simulink model "Read_OpticalFlow_Record"  (R2021b)
settings: Solver=ode2  StartTime=0.0  StopTime=inf  FixedStep=0.001  RelTol=1e-3  EnableMultiTasking=on
model workspace (MAT data in the model file):
  target_system = 1
undefined symbols (not defined in the file): gcbh, JPEG, qc_get_step_size, Video3D, video_display_show
libraries: quarc_library x29
settings Model: SimulationMode=external  ExtModeTrigDuration=10000  Creator=dmadill  LastModifiedBy=user
settings SolverCC: AlgebraicLoopSolver=TrustRegion  PositivePriorityOrder=on
settings DataIOCC: LimitDataPoints=on  SaveFormat=Array  ReturnWorkspaceOutputs=off
settings DebuggingCC: SolverPrmCheckMsg=warning  SFUnexpectedBacktrackingDiag=warning  SFNoUnconditionalDefaultTransitionDiag=warning  SFExecutionAtInitializationDiag=none  SFMachineParentedDataDiag=warning  ArithmeticOperatorsInVariantConditions=warning
settings HardwareCC: ProdBitPerLong=64  ProdHWDeviceType=Intel->x86-64 (Linux 64)
settings ModelReferenceCC: PropagateSignalLabelsOutOfModel=off
settings SFSimCC: SimUseLocalCustomCode=off  CustomCodeUndefinedFunction=UseInterfaceOnly
settings RTWCC: Description=QUARC Linux x64 Target (QDrone) Using Toolchain  SystemTargetFile=quarc_linux_x64.tlc  TemplateMakefile=quarc_default_tmf  RTWUseLocalCustomCode=off  Toolchain=QUARC linux_x64 | gmake (64-bit Windows)  BuildConfiguration=Faster Runs
settings CodeAppCC: StateflowObjectComments=on
settings STFCustomTargetCC: ConcurrentExecutionCompliant=on  UseToolchainInfoCompliant=on  SystemTargetFile=quarc_linux_x64.tlc
settings GRTTargetCC: TargetLangStandard=C89/C90 (ANSI)  ParMdlRefBuildCompliant=off  CompOptLevelCompliant=off  CombineOutputUpdateFcns=off  MatFileLogging=off  CPPClassGenCompliant=off  GRTInterface=on  ExtMode=on  ExtModeMexFile=quarc_comm  ExtModeMexArgs='-w -d /tmp -uri %u', 'tcpip://192.168.2.15:17002?retries=10'
settings ConfigComp: CovMetricSettings=dw  CovSaveCumulativeToWorkspaceVar=on  CovSaveSingleToWorkspaceVar=on  CovExternalEMLEnable=off  CovSFcnEnable=off

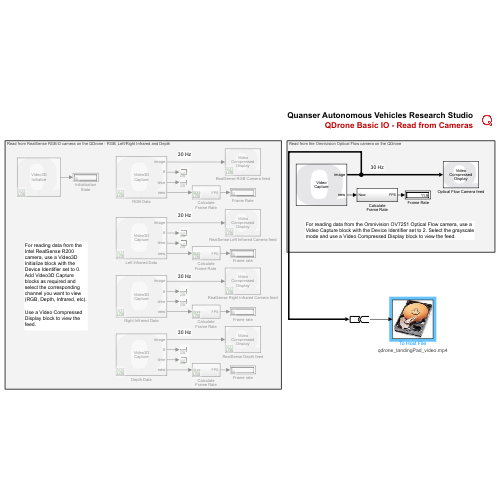
[thumbnail: Simulink's stored preview of the top-level diagram]
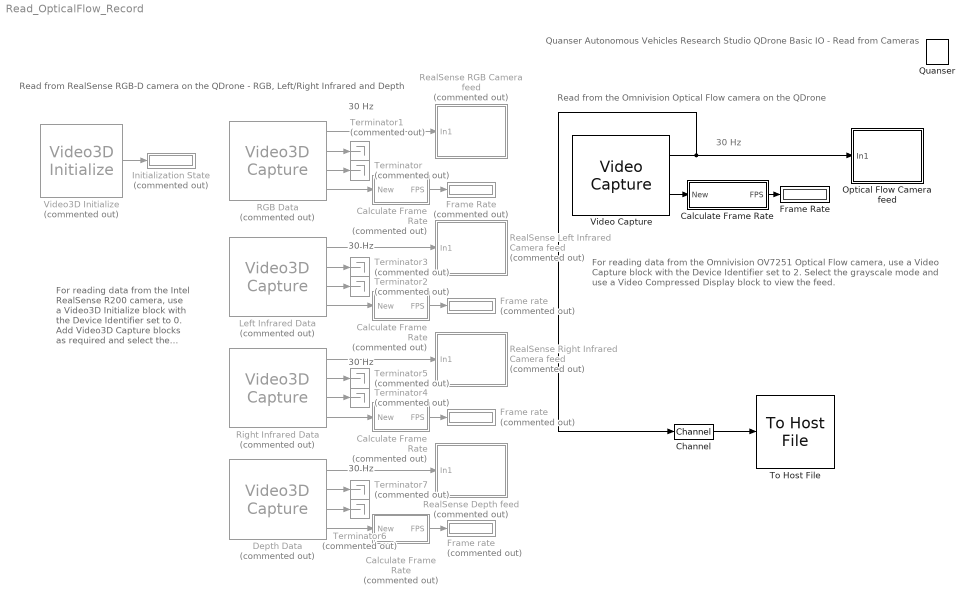
== system Read_OpticalFlow_Record ==
  note: 30 Hz
  note: For reading data from the Omnivision OV7251 Optical Flow camera, use a
      | Video Capture block with the Device Identifier set to 2. Select the grayscale
      | mode and use a Video Compressed Display block to view the feed.
  note: For reading data from the Intel RealSense R200 camera, use a Video3D Initialize block with the Device Identifier set to 0. Add Video3D Capture blocks as required and select the corresponding channel you want to view (RGB, Depth, Infrared, etc).
      |
      | Use a Video Compressed Display block to view the feed.
  note: Read from the Omnivision Optical Flow camera on the QDrone
  note: Read from RealSense RGB-D camera on the QDrone - RGB, Left/Right Infrared and Depth
  note: Quanser Autonomous Vehicles Research Studio
      | QDrone Basic IO - Read from Cameras
  note: 30 Hz
  note: 30 Hz
  note: 30 Hz
  note: 30 Hz
  "   Frame rate   " : Display  Commented=on
  "  Frame Rate " : Display
  "  Frame rate  " : Display  Commented=on
  " Calculate Frame Rate" : Subsystem
  " Frame rate " : Display  Commented=on
  "Calculate Frame Rate  " : Subsystem  Commented=on
  "Calculate Frame Rate " : Subsystem  Commented=on
  Calculate Frame Rate : Subsystem  Commented=on
  "Calculate Frame Rate " : Subsystem  Commented=on
  Channel : quarc_library/Signal Routing/Channel  channel=0  buffer_size=1
  Depth Data : quarc_library/Multimedia/Video3D Capture  Commented=on  object_name=unassigned  stream_type=Depth  stream_index=0  resolution=640 x 480  width=640  height=480  output_format=MATLAB greyscale (HxW)  data_type=uint16  sample_time=qc_get_step_size * ceil(0.033 / qc_get_step_size)  camera_intrinsics=off  depth_scale=off  brightness_override=off  brightness=50.0  contrast_override=off  contrast=50.0  hue_override=off  hue=50.0  saturation_override=off  saturation=50.0  sharpness_override=off  sharpness=50.0  gamma_override=off  gamma=50.0  gain_override=off  gain=50.0  backlightcompensation_override=off  backlightcompensation=50.0  whitebalance_override=Automatic white balance  whitebalance=50.0  exposure_override=Automatic exposure  exposure=30.0  emitter=Enable laser emitter  preset=Do not set camera presets
  Frame Rate : Display  Commented=on
  Initialization State : Display  Commented=on
  Left Infrared Data : quarc_library/Multimedia/Video3D Capture  Commented=on  object_name=unassigned  stream_type=Infrared  stream_index=0  resolution=640 x 480  width=640  height=480  output_format=MATLAB greyscale (HxW)  data_type=uint8  sample_time=qc_get_step_size * ceil(0.033 / qc_get_step_size)  camera_intrinsics=off  depth_scale=off  brightness_override=off  brightness=50.0  contrast_override=off  contrast=50.0  hue_override=off  hue=50.0  saturation_override=off  saturation=50.0  sharpness_override=off  sharpness=50.0  gamma_override=off  gamma=50.0  gain_override=off  gain=50.0  backlightcompensation_override=off  backlightcompensation=50.0  whitebalance_override=Automatic white balance  whitebalance=50.0  exposure_override=Automatic exposure  exposure=30.0  emitter=Enable laser emitter  preset=Do not set camera presets
  Optical Flow Camera feed : Subsystem  LoadFcn=set_param(gcbh, 'UserData', gcb);  StartFcn=video_display_show([gcb, '/Video Display'], 'add', gcb);  mask(Video Compressed Display){algorithm=JPEG, quality=50, sample_time=-1, use_hardware=on}
      mask prompts: algorithm "Compression algorithm:"; quality "Compression quality (0-100):"; sample_time "Sample time (seconds):"; use_hardware "Use hardware acceleration for video display"
      mask help: Displays a video stream on the host, using compression to minimize bandwidth.
      mask init:
      | qc_set_display('Video\nCompressed\nDisplay');
      settings: UndoDeleteFcn=set_param(gcbh, 'UserData', gcb);  OpenFcn=video_display_show([gcb, '/Video Display'], 'show', gcb);  PreDeleteFcn=video_display_show([gcb, '/Video Display'], 'delete');
      settings: CopyFcn=|
      | set_param(gcbh, 'UserData', gcb);
      | set_param(gcbh, 'LinkStatus', 'none');
      settings: NameChangeFcn=|
      | video_display_show([get_param(gcbh, 'UserData'), '/Video Display'], 'rename', [gcb, '/Video Display']);
      | video_display_show([gcb, '/Video Display'], 'add', gcb);
      | set_param(gcbh, 'UserData', gcb);
      mask Help: web(qc_get_block_help_path(gcb));
      mask TypeOptions algorithm: Image Compress/algorithm
      mask TypeOptions quality: Image Compress/quality
      mask TypeOptions sample_time: Video Display/sample_time
      mask TypeOptions use_hardware: Video Display/use_hardware
      mask Display:
      | patch([0.98591 0.98591 0.62618 0.59072 0.56147   0.536   0.536  0.5441 0.56912 0.59207 0.60881 0.62276 0.63527 0.64364  0.6485  0.6485 0.64706 0.64499 0.63662 0.62411 0.61232 0.59837 0.58307 0.56147   0.536   0.536  0.5441  0.5747 0.60953 0.63662 0.67001  0.7034 0.72851 0.75425 0.77927 0.80294 0.82454 0.84119 0.85865 0.87395 0.88574 0.89339  0.8969 0.89969 0.89969 0.89267  0.8816 0.87044 0.85649  0.8384 0.81824 0.80294 0.78764 0.77513 0.76676 0.75776 0.76397 0.77513 0.79178 0.80987 0.82796 0.84326 0.86207 0.98528],[0.18689 0.05522 0.05522 0.05171 0.05171    0.05 0.18338 0.18338 0.19148 0.20435 0.22298 0.24863 0.28589 0.33125 0.38138 0.55139 0.59801 0.63761 0.68189 0.72149 0.74939 0.76694 0.77855 0.79367 0.79952 0.92768 0.92768 0.92768 0.92417 0.92066 0.91364  0.9032 0.89384 0.88106 0.86594 0.85073 0.82634 0.80537 0.77855 0.74363 0.70403 0.65858 0.61079 0.59099 0.41513 0.37202 0.31847 0.29048 0.25556 0.23342  0.2102 0.19382 0.18221 0.17285 0.16943 0.16124  0.1589 0.16241 0.16709 0.17168  0.1787 0.18221 0.18689 0.18689],[0.9,0.90,0.91])
      | patch([0.536 0.52601 0.46823 0.44528 0.41603 0.39101 0.35555 0.33116 0.31451 0.29291  0.2804 0.26717 0.25322 0.23999 0.22406 0.20732 0.19337 0.17528 0.15935 0.14396 0.13217 0.11759 0.10922 0.10085 0.09671 0.09392 0.09041 0.08906 0.08906 0.09464  0.0995 0.10778 0.11894 0.13145 0.14675 0.16349 0.17672 0.19409 0.20732 0.22406 0.23999 0.26159 0.27833 0.29849 0.31793 0.33602 0.35411 0.37085 0.39245 0.41603   0.536   0.536 0.53159 0.46409   0.446 0.42026 0.39587 0.37571 0.36113 0.34925 0.34088 0.33809 0.33809 0.34088 0.34583 0.35627 0.36392 0.38129 0.39587 0.41117 0.42719 0.44672  0.4676 0.48353 0.48353 0.52394   0.536],[0.05 0.04829 0.04712 0.04712 0.04829 0.05063 0.05405 0.05873 0.06107 0.06692 0.07043 0.07619 0.08087 0.08672 0.09482 0.10652 0.11696 0.13325  0.1508 0.17168 0.19499 0.22415 0.25439 0.28472 0.31379 0.35456 0.38489 0.41513 0.58055 0.63878 0.68774 0.72149 0.75641 0.78089 0.80537 0.82859 0.84029 0.85658 0.86594 0.87404  0.8834 0.89267 0.90086 0.90788 0.91247 0.91832 0.92066   0.923 0.92651 0.92768 0.92768 0.79952 0.79952 0.79952 0.79718 0.78899 0.77153 0.75056 0.72149 0.68072 0.62249  0.5549 0.41396 0.37085 0.33242 0.28121 0.25205 0.22181 0.20552 0.19499 0.18572 0.18221 0.17753 0.17636 0.17753  0.1787  0.1787],[0.9,0.90,0.91])
      | disp('Video\nCompressed\nDisplay');
  Quanser : quarc_library/Logos/Quanser
  RGB Data : quarc_library/Multimedia/Video3D Capture  Commented=on  object_name=unassigned  stream_type=RGB  stream_index=0  resolution=640 x 480  width=640  height=480  output_format=MATLAB RGB (HxWx3)  data_type=uint8  sample_time=qc_get_step_size * ceil(0.033 / qc_get_step_size)  camera_intrinsics=off  depth_scale=off  brightness_override=off  brightness=50.0  contrast_override=off  contrast=50.0  hue_override=off  hue=50.0  saturation_override=off  saturation=50.0  sharpness_override=off  sharpness=50.0  gamma_override=off  gamma=50.0  gain_override=off  gain=50.0  backlightcompensation_override=off  backlightcompensation=50.0  whitebalance_override=Automatic white balance  whitebalance=50.0  exposure_override=Automatic exposure  exposure=30.0  emitter=Enable laser emitter  preset=Do not set camera presets
  RealSense Depth feed : Subsystem  Commented=on  LoadFcn=set_param(gcbh, 'UserData', gcb);  StartFcn=video_display_show([gcb, '/Video Display'], 'add', gcb);  mask(Video Compressed Display){algorithm=JPEG, quality=50, sample_time=-1, use_hardware=on}
      mask prompts: algorithm "Compression algorithm:"; quality "Compression quality (0-100):"; sample_time "Sample time (seconds):"; use_hardware "Use hardware acceleration for video display"
      mask help: Displays a video stream on the host, using compression to minimize bandwidth.
      mask init:
      | qc_set_display('Video\nCompressed\nDisplay');
      settings: UndoDeleteFcn=set_param(gcbh, 'UserData', gcb);  OpenFcn=video_display_show([gcb, '/Video Display'], 'show', gcb);  PreDeleteFcn=video_display_show([gcb, '/Video Display'], 'delete');
      settings: CopyFcn=|
      | set_param(gcbh, 'UserData', gcb);
      | set_param(gcbh, 'LinkStatus', 'none');
      settings: NameChangeFcn=|
      | video_display_show([get_param(gcbh, 'UserData'), '/Video Display'], 'rename', [gcb, '/Video Display']);
      | video_display_show([gcb, '/Video Display'], 'add', gcb);
      | set_param(gcbh, 'UserData', gcb);
      mask Help: web(qc_get_block_help_path(gcb));
      mask TypeOptions algorithm: Image Compress/algorithm
      mask TypeOptions quality: Image Compress/quality
      mask TypeOptions sample_time: Video Display/sample_time
      mask TypeOptions use_hardware: Video Display/use_hardware
      mask Display:
      | patch([0.98591 0.98591 0.62618 0.59072 0.56147   0.536   0.536  0.5441 0.56912 0.59207 0.60881 0.62276 0.63527 0.64364  0.6485  0.6485 0.64706 0.64499 0.63662 0.62411 0.61232 0.59837 0.58307 0.56147   0.536   0.536  0.5441  0.5747 0.60953 0.63662 0.67001  0.7034 0.72851 0.75425 0.77927 0.80294 0.82454 0.84119 0.85865 0.87395 0.88574 0.89339  0.8969 0.89969 0.89969 0.89267  0.8816 0.87044 0.85649  0.8384 0.81824 0.80294 0.78764 0.77513 0.76676 0.75776 0.76397 0.77513 0.79178 0.80987 0.82796 0.84326 0.86207 0.98528],[0.18689 0.05522 0.05522 0.05171 0.05171    0.05 0.18338 0.18338 0.19148 0.20435 0.22298 0.24863 0.28589 0.33125 0.38138 0.55139 0.59801 0.63761 0.68189 0.72149 0.74939 0.76694 0.77855 0.79367 0.79952 0.92768 0.92768 0.92768 0.92417 0.92066 0.91364  0.9032 0.89384 0.88106 0.86594 0.85073 0.82634 0.80537 0.77855 0.74363 0.70403 0.65858 0.61079 0.59099 0.41513 0.37202 0.31847 0.29048 0.25556 0.23342  0.2102 0.19382 0.18221 0.17285 0.16943 0.16124  0.1589 0.16241 0.16709 0.17168  0.1787 0.18221 0.18689 0.18689],[0.9,0.90,0.91])
      | patch([0.536 0.52601 0.46823 0.44528 0.41603 0.39101 0.35555 0.33116 0.31451 0.29291  0.2804 0.26717 0.25322 0.23999 0.22406 0.20732 0.19337 0.17528 0.15935 0.14396 0.13217 0.11759 0.10922 0.10085 0.09671 0.09392 0.09041 0.08906 0.08906 0.09464  0.0995 0.10778 0.11894 0.13145 0.14675 0.16349 0.17672 0.19409 0.20732 0.22406 0.23999 0.26159 0.27833 0.29849 0.31793 0.33602 0.35411 0.37085 0.39245 0.41603   0.536   0.536 0.53159 0.46409   0.446 0.42026 0.39587 0.37571 0.36113 0.34925 0.34088 0.33809 0.33809 0.34088 0.34583 0.35627 0.36392 0.38129 0.39587 0.41117 0.42719 0.44672  0.4676 0.48353 0.48353 0.52394   0.536],[0.05 0.04829 0.04712 0.04712 0.04829 0.05063 0.05405 0.05873 0.06107 0.06692 0.07043 0.07619 0.08087 0.08672 0.09482 0.10652 0.11696 0.13325  0.1508 0.17168 0.19499 0.22415 0.25439 0.28472 0.31379 0.35456 0.38489 0.41513 0.58055 0.63878 0.68774 0.72149 0.75641 0.78089 0.80537 0.82859 0.84029 0.85658 0.86594 0.87404  0.8834 0.89267 0.90086 0.90788 0.91247 0.91832 0.92066   0.923 0.92651 0.92768 0.92768 0.79952 0.79952 0.79952 0.79718 0.78899 0.77153 0.75056 0.72149 0.68072 0.62249  0.5549 0.41396 0.37085 0.33242 0.28121 0.25205 0.22181 0.20552 0.19499 0.18572 0.18221 0.17753 0.17636 0.17753  0.1787  0.1787],[0.9,0.90,0.91])
      | disp('Video\nCompressed\nDisplay');
  RealSense Left Infrared Camera feed : Subsystem  Commented=on  LoadFcn=set_param(gcbh, 'UserData', gcb);  StartFcn=video_display_show([gcb, '/Video Display'], 'add', gcb);  mask(Video Compressed Display){algorithm=JPEG, quality=50, sample_time=-1, use_hardware=on}
      mask prompts: algorithm "Compression algorithm:"; quality "Compression quality (0-100):"; sample_time "Sample time (seconds):"; use_hardware "Use hardware acceleration for video display"
      mask help: Displays a video stream on the host, using compression to minimize bandwidth.
      mask init:
      | qc_set_display('Video\nCompressed\nDisplay');
      settings: UndoDeleteFcn=set_param(gcbh, 'UserData', gcb);  OpenFcn=video_display_show([gcb, '/Video Display'], 'show', gcb);  PreDeleteFcn=video_display_show([gcb, '/Video Display'], 'delete');
      settings: CopyFcn=|
      | set_param(gcbh, 'UserData', gcb);
      | set_param(gcbh, 'LinkStatus', 'none');
      settings: NameChangeFcn=|
      | video_display_show([get_param(gcbh, 'UserData'), '/Video Display'], 'rename', [gcb, '/Video Display']);
      | video_display_show([gcb, '/Video Display'], 'add', gcb);
      | set_param(gcbh, 'UserData', gcb);
      mask Help: web(qc_get_block_help_path(gcb));
      mask TypeOptions algorithm: Image Compress/algorithm
      mask TypeOptions quality: Image Compress/quality
      mask TypeOptions sample_time: Video Display/sample_time
      mask TypeOptions use_hardware: Video Display/use_hardware
      mask Display:
      | patch([0.98591 0.98591 0.62618 0.59072 0.56147   0.536   0.536  0.5441 0.56912 0.59207 0.60881 0.62276 0.63527 0.64364  0.6485  0.6485 0.64706 0.64499 0.63662 0.62411 0.61232 0.59837 0.58307 0.56147   0.536   0.536  0.5441  0.5747 0.60953 0.63662 0.67001  0.7034 0.72851 0.75425 0.77927 0.80294 0.82454 0.84119 0.85865 0.87395 0.88574 0.89339  0.8969 0.89969 0.89969 0.89267  0.8816 0.87044 0.85649  0.8384 0.81824 0.80294 0.78764 0.77513 0.76676 0.75776 0.76397 0.77513 0.79178 0.80987 0.82796 0.84326 0.86207 0.98528],[0.18689 0.05522 0.05522 0.05171 0.05171    0.05 0.18338 0.18338 0.19148 0.20435 0.22298 0.24863 0.28589 0.33125 0.38138 0.55139 0.59801 0.63761 0.68189 0.72149 0.74939 0.76694 0.77855 0.79367 0.79952 0.92768 0.92768 0.92768 0.92417 0.92066 0.91364  0.9032 0.89384 0.88106 0.86594 0.85073 0.82634 0.80537 0.77855 0.74363 0.70403 0.65858 0.61079 0.59099 0.41513 0.37202 0.31847 0.29048 0.25556 0.23342  0.2102 0.19382 0.18221 0.17285 0.16943 0.16124  0.1589 0.16241 0.16709 0.17168  0.1787 0.18221 0.18689 0.18689],[0.9,0.90,0.91])
      | patch([0.536 0.52601 0.46823 0.44528 0.41603 0.39101 0.35555 0.33116 0.31451 0.29291  0.2804 0.26717 0.25322 0.23999 0.22406 0.20732 0.19337 0.17528 0.15935 0.14396 0.13217 0.11759 0.10922 0.10085 0.09671 0.09392 0.09041 0.08906 0.08906 0.09464  0.0995 0.10778 0.11894 0.13145 0.14675 0.16349 0.17672 0.19409 0.20732 0.22406 0.23999 0.26159 0.27833 0.29849 0.31793 0.33602 0.35411 0.37085 0.39245 0.41603   0.536   0.536 0.53159 0.46409   0.446 0.42026 0.39587 0.37571 0.36113 0.34925 0.34088 0.33809 0.33809 0.34088 0.34583 0.35627 0.36392 0.38129 0.39587 0.41117 0.42719 0.44672  0.4676 0.48353 0.48353 0.52394   0.536],[0.05 0.04829 0.04712 0.04712 0.04829 0.05063 0.05405 0.05873 0.06107 0.06692 0.07043 0.07619 0.08087 0.08672 0.09482 0.10652 0.11696 0.13325  0.1508 0.17168 0.19499 0.22415 0.25439 0.28472 0.31379 0.35456 0.38489 0.41513 0.58055 0.63878 0.68774 0.72149 0.75641 0.78089 0.80537 0.82859 0.84029 0.85658 0.86594 0.87404  0.8834 0.89267 0.90086 0.90788 0.91247 0.91832 0.92066   0.923 0.92651 0.92768 0.92768 0.79952 0.79952 0.79952 0.79718 0.78899 0.77153 0.75056 0.72149 0.68072 0.62249  0.5549 0.41396 0.37085 0.33242 0.28121 0.25205 0.22181 0.20552 0.19499 0.18572 0.18221 0.17753 0.17636 0.17753  0.1787  0.1787],[0.9,0.90,0.91])
      | disp('Video\nCompressed\nDisplay');
  RealSense RGB Camera feed : Subsystem  Commented=on  LoadFcn=set_param(gcbh, 'UserData', gcb);  StartFcn=video_display_show([gcb, '/Video Display'], 'add', gcb);  mask(Video Compressed Display){algorithm=JPEG, quality=50, sample_time=-1, use_hardware=on}
      mask prompts: algorithm "Compression algorithm:"; quality "Compression quality (0-100):"; sample_time "Sample time (seconds):"; use_hardware "Use hardware acceleration for video display"
      mask help: Displays a video stream on the host, using compression to minimize bandwidth.
      mask init:
      | qc_set_display('Video\nCompressed\nDisplay');
      settings: UndoDeleteFcn=set_param(gcbh, 'UserData', gcb);  OpenFcn=video_display_show([gcb, '/Video Display'], 'show', gcb);  PreDeleteFcn=video_display_show([gcb, '/Video Display'], 'delete');
      settings: CopyFcn=|
      | set_param(gcbh, 'UserData', gcb);
      | set_param(gcbh, 'LinkStatus', 'none');
      settings: NameChangeFcn=|
      | video_display_show([get_param(gcbh, 'UserData'), '/Video Display'], 'rename', [gcb, '/Video Display']);
      | video_display_show([gcb, '/Video Display'], 'add', gcb);
      | set_param(gcbh, 'UserData', gcb);
      mask Help: web(qc_get_block_help_path(gcb));
      mask TypeOptions algorithm: Image Compress/algorithm
      mask TypeOptions quality: Image Compress/quality
      mask TypeOptions sample_time: Video Display/sample_time
      mask TypeOptions use_hardware: Video Display/use_hardware
      mask Display:
      | patch([0.98591 0.98591 0.62618 0.59072 0.56147   0.536   0.536  0.5441 0.56912 0.59207 0.60881 0.62276 0.63527 0.64364  0.6485  0.6485 0.64706 0.64499 0.63662 0.62411 0.61232 0.59837 0.58307 0.56147   0.536   0.536  0.5441  0.5747 0.60953 0.63662 0.67001  0.7034 0.72851 0.75425 0.77927 0.80294 0.82454 0.84119 0.85865 0.87395 0.88574 0.89339  0.8969 0.89969 0.89969 0.89267  0.8816 0.87044 0.85649  0.8384 0.81824 0.80294 0.78764 0.77513 0.76676 0.75776 0.76397 0.77513 0.79178 0.80987 0.82796 0.84326 0.86207 0.98528],[0.18689 0.05522 0.05522 0.05171 0.05171    0.05 0.18338 0.18338 0.19148 0.20435 0.22298 0.24863 0.28589 0.33125 0.38138 0.55139 0.59801 0.63761 0.68189 0.72149 0.74939 0.76694 0.77855 0.79367 0.79952 0.92768 0.92768 0.92768 0.92417 0.92066 0.91364  0.9032 0.89384 0.88106 0.86594 0.85073 0.82634 0.80537 0.77855 0.74363 0.70403 0.65858 0.61079 0.59099 0.41513 0.37202 0.31847 0.29048 0.25556 0.23342  0.2102 0.19382 0.18221 0.17285 0.16943 0.16124  0.1589 0.16241 0.16709 0.17168  0.1787 0.18221 0.18689 0.18689],[0.9,0.90,0.91])
      | patch([0.536 0.52601 0.46823 0.44528 0.41603 0.39101 0.35555 0.33116 0.31451 0.29291  0.2804 0.26717 0.25322 0.23999 0.22406 0.20732 0.19337 0.17528 0.15935 0.14396 0.13217 0.11759 0.10922 0.10085 0.09671 0.09392 0.09041 0.08906 0.08906 0.09464  0.0995 0.10778 0.11894 0.13145 0.14675 0.16349 0.17672 0.19409 0.20732 0.22406 0.23999 0.26159 0.27833 0.29849 0.31793 0.33602 0.35411 0.37085 0.39245 0.41603   0.536   0.536 0.53159 0.46409   0.446 0.42026 0.39587 0.37571 0.36113 0.34925 0.34088 0.33809 0.33809 0.34088 0.34583 0.35627 0.36392 0.38129 0.39587 0.41117 0.42719 0.44672  0.4676 0.48353 0.48353 0.52394   0.536],[0.05 0.04829 0.04712 0.04712 0.04829 0.05063 0.05405 0.05873 0.06107 0.06692 0.07043 0.07619 0.08087 0.08672 0.09482 0.10652 0.11696 0.13325  0.1508 0.17168 0.19499 0.22415 0.25439 0.28472 0.31379 0.35456 0.38489 0.41513 0.58055 0.63878 0.68774 0.72149 0.75641 0.78089 0.80537 0.82859 0.84029 0.85658 0.86594 0.87404  0.8834 0.89267 0.90086 0.90788 0.91247 0.91832 0.92066   0.923 0.92651 0.92768 0.92768 0.79952 0.79952 0.79952 0.79718 0.78899 0.77153 0.75056 0.72149 0.68072 0.62249  0.5549 0.41396 0.37085 0.33242 0.28121 0.25205 0.22181 0.20552 0.19499 0.18572 0.18221 0.17753 0.17636 0.17753  0.1787  0.1787],[0.9,0.90,0.91])
      | disp('Video\nCompressed\nDisplay');
  RealSense Right Infrared Camera feed : Subsystem  Commented=on  LoadFcn=set_param(gcbh, 'UserData', gcb);  StartFcn=video_display_show([gcb, '/Video Display'], 'add', gcb);  mask(Video Compressed Display){algorithm=JPEG, quality=50, sample_time=-1, use_hardware=on}
      mask prompts: algorithm "Compression algorithm:"; quality "Compression quality (0-100):"; sample_time "Sample time (seconds):"; use_hardware "Use hardware acceleration for video display"
      mask help: Displays a video stream on the host, using compression to minimize bandwidth.
      mask init:
      | qc_set_display('Video\nCompressed\nDisplay');
      settings: UndoDeleteFcn=set_param(gcbh, 'UserData', gcb);  OpenFcn=video_display_show([gcb, '/Video Display'], 'show', gcb);  PreDeleteFcn=video_display_show([gcb, '/Video Display'], 'delete');
      settings: CopyFcn=|
      | set_param(gcbh, 'UserData', gcb);
      | set_param(gcbh, 'LinkStatus', 'none');
      settings: NameChangeFcn=|
      | video_display_show([get_param(gcbh, 'UserData'), '/Video Display'], 'rename', [gcb, '/Video Display']);
      | video_display_show([gcb, '/Video Display'], 'add', gcb);
      | set_param(gcbh, 'UserData', gcb);
      mask Help: web(qc_get_block_help_path(gcb));
      mask TypeOptions algorithm: Image Compress/algorithm
      mask TypeOptions quality: Image Compress/quality
      mask TypeOptions sample_time: Video Display/sample_time
      mask TypeOptions use_hardware: Video Display/use_hardware
      mask Display:
      | patch([0.98591 0.98591 0.62618 0.59072 0.56147   0.536   0.536  0.5441 0.56912 0.59207 0.60881 0.62276 0.63527 0.64364  0.6485  0.6485 0.64706 0.64499 0.63662 0.62411 0.61232 0.59837 0.58307 0.56147   0.536   0.536  0.5441  0.5747 0.60953 0.63662 0.67001  0.7034 0.72851 0.75425 0.77927 0.80294 0.82454 0.84119 0.85865 0.87395 0.88574 0.89339  0.8969 0.89969 0.89969 0.89267  0.8816 0.87044 0.85649  0.8384 0.81824 0.80294 0.78764 0.77513 0.76676 0.75776 0.76397 0.77513 0.79178 0.80987 0.82796 0.84326 0.86207 0.98528],[0.18689 0.05522 0.05522 0.05171 0.05171    0.05 0.18338 0.18338 0.19148 0.20435 0.22298 0.24863 0.28589 0.33125 0.38138 0.55139 0.59801 0.63761 0.68189 0.72149 0.74939 0.76694 0.77855 0.79367 0.79952 0.92768 0.92768 0.92768 0.92417 0.92066 0.91364  0.9032 0.89384 0.88106 0.86594 0.85073 0.82634 0.80537 0.77855 0.74363 0.70403 0.65858 0.61079 0.59099 0.41513 0.37202 0.31847 0.29048 0.25556 0.23342  0.2102 0.19382 0.18221 0.17285 0.16943 0.16124  0.1589 0.16241 0.16709 0.17168  0.1787 0.18221 0.18689 0.18689],[0.9,0.90,0.91])
      | patch([0.536 0.52601 0.46823 0.44528 0.41603 0.39101 0.35555 0.33116 0.31451 0.29291  0.2804 0.26717 0.25322 0.23999 0.22406 0.20732 0.19337 0.17528 0.15935 0.14396 0.13217 0.11759 0.10922 0.10085 0.09671 0.09392 0.09041 0.08906 0.08906 0.09464  0.0995 0.10778 0.11894 0.13145 0.14675 0.16349 0.17672 0.19409 0.20732 0.22406 0.23999 0.26159 0.27833 0.29849 0.31793 0.33602 0.35411 0.37085 0.39245 0.41603   0.536   0.536 0.53159 0.46409   0.446 0.42026 0.39587 0.37571 0.36113 0.34925 0.34088 0.33809 0.33809 0.34088 0.34583 0.35627 0.36392 0.38129 0.39587 0.41117 0.42719 0.44672  0.4676 0.48353 0.48353 0.52394   0.536],[0.05 0.04829 0.04712 0.04712 0.04829 0.05063 0.05405 0.05873 0.06107 0.06692 0.07043 0.07619 0.08087 0.08672 0.09482 0.10652 0.11696 0.13325  0.1508 0.17168 0.19499 0.22415 0.25439 0.28472 0.31379 0.35456 0.38489 0.41513 0.58055 0.63878 0.68774 0.72149 0.75641 0.78089 0.80537 0.82859 0.84029 0.85658 0.86594 0.87404  0.8834 0.89267 0.90086 0.90788 0.91247 0.91832 0.92066   0.923 0.92651 0.92768 0.92768 0.79952 0.79952 0.79952 0.79718 0.78899 0.77153 0.75056 0.72149 0.68072 0.62249  0.5549 0.41396 0.37085 0.33242 0.28121 0.25205 0.22181 0.20552 0.19499 0.18572 0.18221 0.17753 0.17636 0.17753  0.1787  0.1787],[0.9,0.90,0.91])
      | disp('Video\nCompressed\nDisplay');
  Right Infrared Data : quarc_library/Multimedia/Video3D Capture  Commented=on  object_name=unassigned  stream_type=Infrared  stream_index=1  resolution=640 x 480  width=640  height=480  output_format=MATLAB greyscale (HxW)  data_type=uint8  sample_time=qc_get_step_size * ceil(0.033 / qc_get_step_size)  camera_intrinsics=off  depth_scale=off  brightness_override=off  brightness=50.0  contrast_override=off  contrast=50.0  hue_override=off  hue=50.0  saturation_override=off  saturation=50.0  sharpness_override=off  sharpness=50.0  gamma_override=off  gamma=50.0  gain_override=off  gain=50.0  backlightcompensation_override=off  backlightcompensation=50.0  whitebalance_override=Automatic white balance  whitebalance=50.0  exposure_override=Automatic exposure  exposure=30.0  emitter=Enable laser emitter  preset=Do not set camera presets
  Terminator{,1..7} (8 alike) : Terminator  Commented=on
  To Host File : quarc_library/Sinks/To Host/To Host File  file_name=qdrone_landingPad_video.mp4  variable_name=data  decimation=1  sample_time=-1  file_format=Video file  options=No header or footer  append=off  final_file_name=qdrone_landingPad_video.mp4  bitrate=2000000
  Video Capture : quarc_library/Multimedia/Video Capture  source=device  device=2  filename=sample_movie.mov  value=[0 0; 0 0]  resolution=640 x 480  width=640  height=480  output_format=MATLAB greyscale (HxW)  data_type=uint8  sample_time=qc_get_step_size * ceil(1/30 / qc_get_step_size)  brightness_override=off  brightness=50.0  contrast_override=off  contrast=50.0  hue_override=off  hue=50.0  saturation_override=off  saturation=50.0  sharpness_override=off  sharpness=50.0  gamma_override=off  gamma=50.0  coloreffect_override=off  coloreffect=None  whitebalance_override=off  whitebalance=50.0  backlightcompensation_override=off  backlightcompensation=0.0  gain_override=off  gain=50.0  pan_override=off  pan=50.0  tilt_override=off  tilt=50.0  roll_override=off  roll=50.0  zoom_override=off  zoom=0.0  exposure_override=off  exposure=50.0  iris_override=off  iris=50.0  focus_override=off  focus=0.0
      settings: SourceProductName=QUARC Targets
  Video3D Initialize : quarc_library/Multimedia/Video3D Initialize  Commented=on  object_name=Video3D-1  source=Device  identifier=0  file=sample.bag  sample_time=qc_get_step_size * ceil(0.033 / qc_get_step_size)  active=on
  wires:
  Calculate Frame Rate/1(FPS) -> Frame Rate/1
  "Calculate Frame Rate "/1(FPS) -> " Frame rate "/1
  RGB Data/4 -> Calculate Frame Rate/1(New)
  RGB Data/1 -> RealSense RGB Camera feed/1(In1)
  RGB Data/3 -> Terminator/1
  RGB Data/2 -> Terminator1/1
  Left Infrared Data/4 -> "Calculate Frame Rate "/1(New)
  Left Infrared Data/1 -> RealSense Left Infrared Camera feed/1(In1)
  Left Infrared Data/2 -> Terminator3/1
  Left Infrared Data/3 -> Terminator2/1
  Right Infrared Data/3 -> Terminator4/1
  Right Infrared Data/2 -> Terminator5/1
  Right Infrared Data/1 -> RealSense Right Infrared Camera feed/1(In1)
  Right Infrared Data/4 -> "Calculate Frame Rate  "/1(New)
  "Calculate Frame Rate  "/1(FPS) -> "  Frame rate  "/1
  "Calculate Frame Rate "/1(FPS) -> "   Frame rate   "/1
  Depth Data/4 -> "Calculate Frame Rate "/1(New)
  Depth Data/1 -> RealSense Depth feed/1(In1)
  Depth Data/2 -> Terminator7/1
  Depth Data/3 -> Terminator6/1
  Video3D Initialize/1 -> Initialization State/1
  Video Capture/2 -> " Calculate Frame Rate"/1(New)
  " Calculate Frame Rate"/1(FPS) -> "  Frame Rate "/1
  Channel/1 -> To Host File/1
  Video Capture/1 -> Channel/1, Optical Flow Camera feed/1(In1)

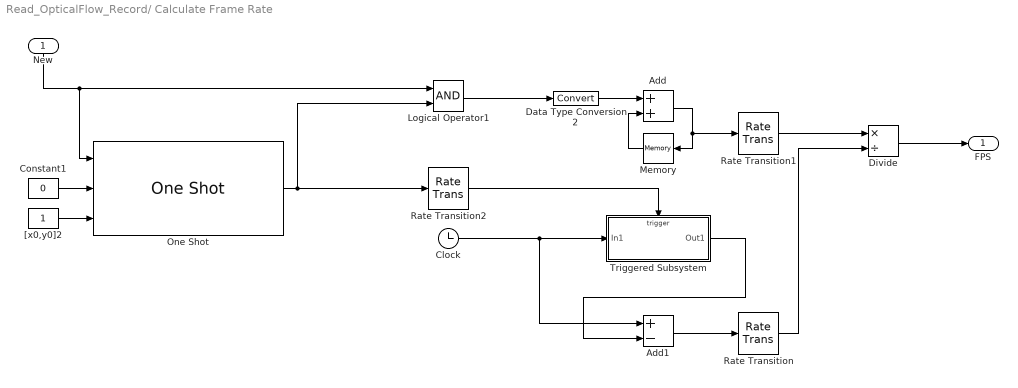
== system Read_OpticalFlow_Record/ Calculate Frame Rate ==
  New : Inport
  Add : Sum
  Add1 : Sum  Inputs=+-
  Clock : Clock
  Constant1 : Constant  Value=0
  Data Type Conversion2 : DataTypeConversion
  Divide : Product  Inputs=*/
  Logical Operator1 : Logic  AllPortsSameDT=off  OutDataTypeStr=boolean
  Memory : Memory  InheritSampleTime=on
  One Shot : quarc_library/Discontinuities/One Shot  trigger_type=Rising edge  redun_pulse=Extend pulse width  width_source=Specify via dialog  pulse_width=1000
      settings: SourceProductName=QUARC Targets
  Rate Transition : RateTransition
  Rate Transition1 : RateTransition
  Rate Transition2 : RateTransition
  Triggered Subsystem : Subsystem  TreatAsAtomicUnit=on
  "[x0,y0]2" : Constant
  FPS : Outport
  wires:
  Divide/1 -> FPS/1
  Rate Transition/1 -> Divide/2
  Clock/1 -> Triggered Subsystem/1(In1), Add1/1
  Add/1 -> Rate Transition1/1, Memory/1
  Memory/1 -> Add/2
  Rate Transition1/1 -> Divide/1
  Triggered Subsystem/1(Out1) -> Add1/2
  New/1 -> Logical Operator1/1, One Shot/1
  Constant1/1 -> One Shot/2
  "[x0,y0]2"/1 -> One Shot/3
  Logical Operator1/1 -> Data Type Conversion2/1
  Data Type Conversion2/1 -> Add/1
  Rate Transition2/1 -> Triggered Subsystem/Trigger
  Add1/1 -> Rate Transition/1
  One Shot/1 -> Logical Operator1/2, Rate Transition2/1

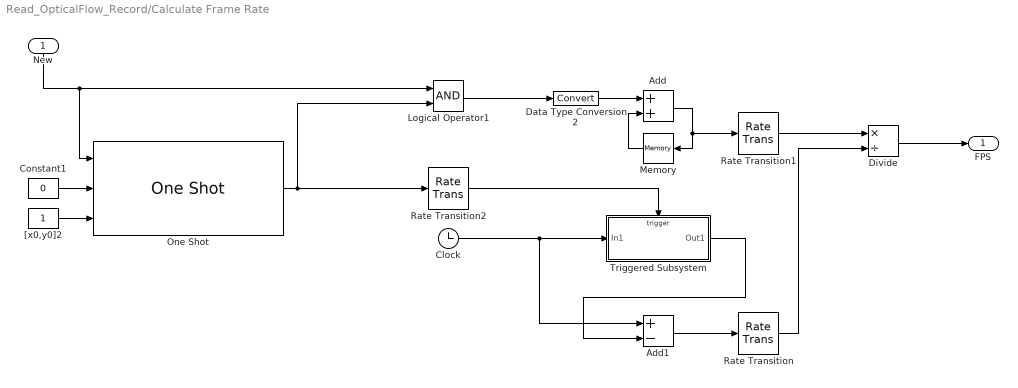
== system Read_OpticalFlow_Record/Calculate Frame Rate   ==
  New : Inport
  Add : Sum
  Add1 : Sum  Inputs=+-
  Clock : Clock
  Constant1 : Constant  Value=0
  Data Type Conversion2 : DataTypeConversion
  Divide : Product  Inputs=*/
  Logical Operator1 : Logic  AllPortsSameDT=off  OutDataTypeStr=boolean
  Memory : Memory  InheritSampleTime=on
  One Shot : quarc_library/Discontinuities/One Shot  trigger_type=Rising edge  redun_pulse=Extend pulse width  width_source=Specify via dialog  pulse_width=1000
      settings: SourceProductName=QUARC Targets
  Rate Transition : RateTransition
  Rate Transition1 : RateTransition
  Rate Transition2 : RateTransition
  Triggered Subsystem : Subsystem  TreatAsAtomicUnit=on
  "[x0,y0]2" : Constant
  FPS : Outport
  wires:
  One Shot/1 -> Rate Transition2/1, Logical Operator1/2
  Add1/1 -> Rate Transition/1
  Rate Transition2/1 -> Triggered Subsystem/Trigger
  Data Type Conversion2/1 -> Add/1
  Logical Operator1/1 -> Data Type Conversion2/1
  "[x0,y0]2"/1 -> One Shot/3
  Constant1/1 -> One Shot/2
  New/1 -> One Shot/1, Logical Operator1/1
  Triggered Subsystem/1(Out1) -> Add1/2
  Rate Transition1/1 -> Divide/1
  Memory/1 -> Add/2
  Add/1 -> Memory/1, Rate Transition1/1
  Clock/1 -> Add1/1, Triggered Subsystem/1(In1)
  Rate Transition/1 -> Divide/2
  Divide/1 -> FPS/1

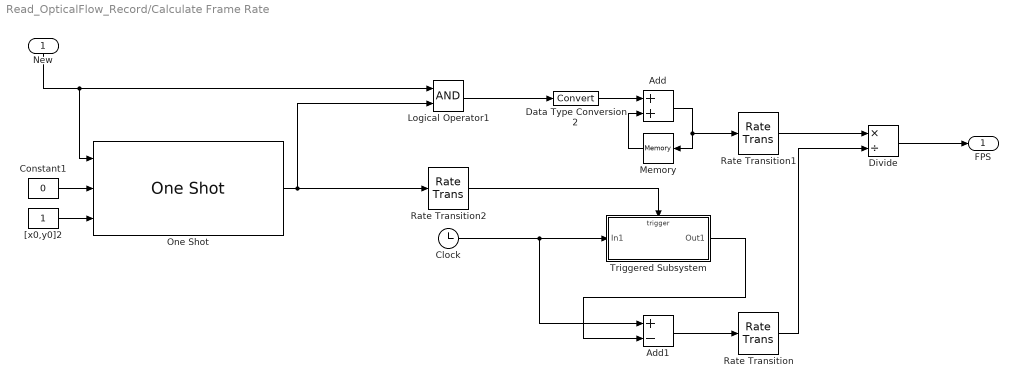
== system Read_OpticalFlow_Record/Calculate Frame Rate  ==
  New : Inport
  Add : Sum
  Add1 : Sum  Inputs=+-
  Clock : Clock
  Constant1 : Constant  Value=0
  Data Type Conversion2 : DataTypeConversion
  Divide : Product  Inputs=*/
  Logical Operator1 : Logic  AllPortsSameDT=off  OutDataTypeStr=boolean
  Memory : Memory  InheritSampleTime=on
  One Shot : quarc_library/Discontinuities/One Shot  trigger_type=Rising edge  redun_pulse=Extend pulse width  width_source=Specify via dialog  pulse_width=1000
      settings: SourceProductName=QUARC Targets
  Rate Transition : RateTransition
  Rate Transition1 : RateTransition
  Rate Transition2 : RateTransition
  Triggered Subsystem : Subsystem  TreatAsAtomicUnit=on
  "[x0,y0]2" : Constant
  FPS : Outport
  wires:
  Divide/1 -> FPS/1
  Rate Transition/1 -> Divide/2
  Clock/1 -> Triggered Subsystem/1(In1), Add1/1
  Add/1 -> Rate Transition1/1, Memory/1
  Memory/1 -> Add/2
  Rate Transition1/1 -> Divide/1
  Triggered Subsystem/1(Out1) -> Add1/2
  New/1 -> Logical Operator1/1, One Shot/1
  Constant1/1 -> One Shot/2
  "[x0,y0]2"/1 -> One Shot/3
  Logical Operator1/1 -> Data Type Conversion2/1
  Data Type Conversion2/1 -> Add/1
  Rate Transition2/1 -> Triggered Subsystem/Trigger
  Add1/1 -> Rate Transition/1
  One Shot/1 -> Logical Operator1/2, Rate Transition2/1

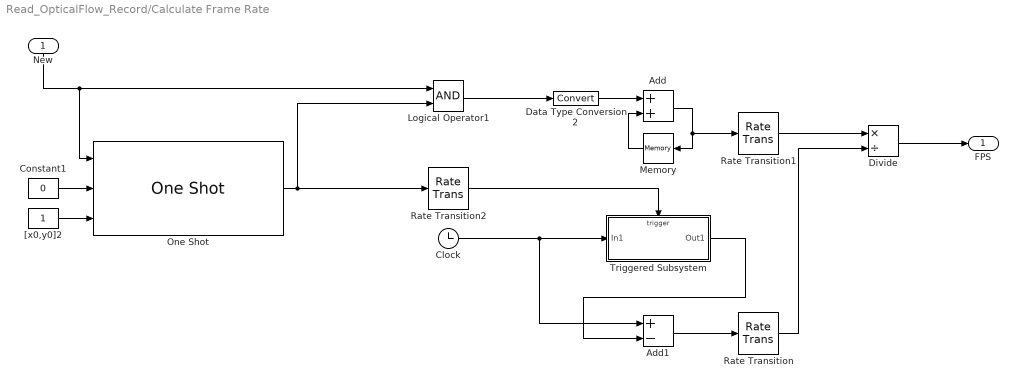
== system Read_OpticalFlow_Record/Calculate Frame Rate ==
  New : Inport
  Add : Sum
  Add1 : Sum  Inputs=+-
  Clock : Clock
  Constant1 : Constant  Value=0
  Data Type Conversion2 : DataTypeConversion
  Divide : Product  Inputs=*/
  Logical Operator1 : Logic  AllPortsSameDT=off  OutDataTypeStr=boolean
  Memory : Memory  InheritSampleTime=on
  One Shot : quarc_library/Discontinuities/One Shot  trigger_type=Rising edge  redun_pulse=Extend pulse width  width_source=Specify via dialog  pulse_width=1000
      settings: SourceProductName=QUARC Targets
  Rate Transition : RateTransition
  Rate Transition1 : RateTransition
  Rate Transition2 : RateTransition
  Triggered Subsystem : Subsystem  TreatAsAtomicUnit=on
  "[x0,y0]2" : Constant
  FPS : Outport
  wires:
  One Shot/1 -> Rate Transition2/1, Logical Operator1/2
  Add1/1 -> Rate Transition/1
  Rate Transition2/1 -> Triggered Subsystem/Trigger
  Data Type Conversion2/1 -> Add/1
  Logical Operator1/1 -> Data Type Conversion2/1
  "[x0,y0]2"/1 -> One Shot/3
  Constant1/1 -> One Shot/2
  New/1 -> One Shot/1, Logical Operator1/1
  Triggered Subsystem/1(Out1) -> Add1/2
  Rate Transition1/1 -> Divide/1
  Memory/1 -> Add/2
  Add/1 -> Memory/1, Rate Transition1/1
  Clock/1 -> Add1/1, Triggered Subsystem/1(In1)
  Rate Transition/1 -> Divide/2
  Divide/1 -> FPS/1

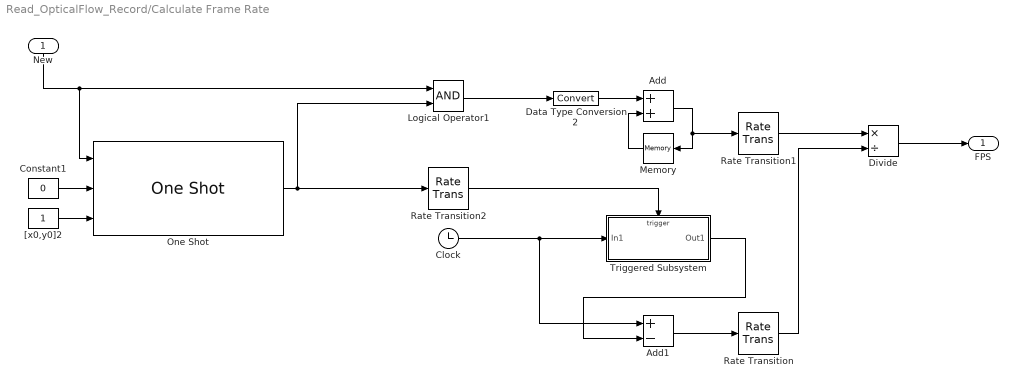
== system Read_OpticalFlow_Record/Calculate Frame Rate  ==
  New : Inport
  Add : Sum
  Add1 : Sum  Inputs=+-
  Clock : Clock
  Constant1 : Constant  Value=0
  Data Type Conversion2 : DataTypeConversion
  Divide : Product  Inputs=*/
  Logical Operator1 : Logic  AllPortsSameDT=off  OutDataTypeStr=boolean
  Memory : Memory  InheritSampleTime=on
  One Shot : quarc_library/Discontinuities/One Shot  trigger_type=Rising edge  redun_pulse=Extend pulse width  width_source=Specify via dialog  pulse_width=1000
      settings: SourceProductName=QUARC Targets
  Rate Transition : RateTransition
  Rate Transition1 : RateTransition
  Rate Transition2 : RateTransition
  Triggered Subsystem : Subsystem  TreatAsAtomicUnit=on
  "[x0,y0]2" : Constant
  FPS : Outport
  wires:
  Divide/1 -> FPS/1
  Rate Transition/1 -> Divide/2
  Clock/1 -> Triggered Subsystem/1(In1), Add1/1
  Add/1 -> Rate Transition1/1, Memory/1
  Memory/1 -> Add/2
  Rate Transition1/1 -> Divide/1
  Triggered Subsystem/1(Out1) -> Add1/2
  New/1 -> Logical Operator1/1, One Shot/1
  Constant1/1 -> One Shot/2
  "[x0,y0]2"/1 -> One Shot/3
  Logical Operator1/1 -> Data Type Conversion2/1
  Data Type Conversion2/1 -> Add/1
  Rate Transition2/1 -> Triggered Subsystem/Trigger
  Add1/1 -> Rate Transition/1
  One Shot/1 -> Logical Operator1/2, Rate Transition2/1

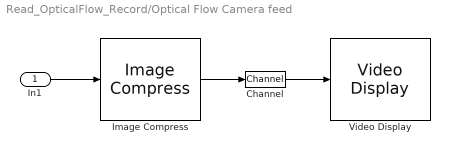
== system Read_OpticalFlow_Record/Optical Flow Camera feed ==
  In1 : Inport
  Channel : quarc_library/Signal Routing/Channel  channel=1  buffer_size=1
  Image Compress : quarc_library/Image Processing/Generic/Image Compress  algorithm=JPEG  source=Internal dialog parameter  quality=quality  output_dim=-1
  Video Display : quarc_library/Multimedia/Video Display  Tag=Read_OpticalFlow_Record/Optical Flow Camera feed/Video Display  sample_time=sample_time  use_hardware=on
  wires:
  Channel/1 -> Video Display/1
  In1/1 -> Image Compress/1
  Image Compress/1 -> Channel/1

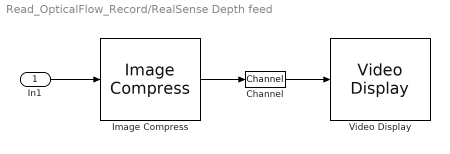
== system Read_OpticalFlow_Record/RealSense Depth feed ==
  In1 : Inport
  Channel : quarc_library/Signal Routing/Channel  channel=2  buffer_size=1
  Image Compress : quarc_library/Image Processing/Generic/Image Compress  algorithm=JPEG  source=Internal dialog parameter  quality=quality  output_dim=-1
  Video Display : quarc_library/Multimedia/Video Display  Tag=Read_OpticalFlow_Record/RealSense Depth feed/Video Display  sample_time=sample_time  use_hardware=on
  wires:
  Channel/1 -> Video Display/1
  In1/1 -> Image Compress/1
  Image Compress/1 -> Channel/1

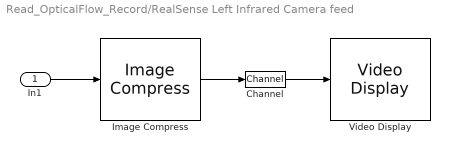
== system Read_OpticalFlow_Record/RealSense Left Infrared Camera feed ==
  In1 : Inport
  Channel : quarc_library/Signal Routing/Channel  channel=3  buffer_size=1
  Image Compress : quarc_library/Image Processing/Generic/Image Compress  algorithm=JPEG  source=Internal dialog parameter  quality=quality  output_dim=-1
  Video Display : quarc_library/Multimedia/Video Display  Tag=Read_OpticalFlow_Record/RealSense Left Infrared Camera feed/Video Display  sample_time=sample_time  use_hardware=on
  wires:
  Channel/1 -> Video Display/1
  In1/1 -> Image Compress/1
  Image Compress/1 -> Channel/1

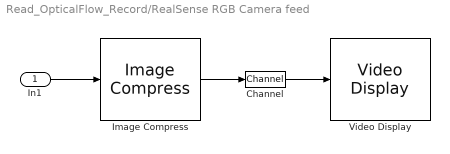
== system Read_OpticalFlow_Record/RealSense RGB Camera feed ==
  In1 : Inport
  Channel : quarc_library/Signal Routing/Channel  channel=4  buffer_size=1
  Image Compress : quarc_library/Image Processing/Generic/Image Compress  algorithm=JPEG  source=Internal dialog parameter  quality=quality  output_dim=-1
  Video Display : quarc_library/Multimedia/Video Display  Tag=Read_OpticalFlow_Record/RealSense RGB Camera feed/Video Display  sample_time=sample_time  use_hardware=on
  wires:
  Image Compress/1 -> Channel/1
  In1/1 -> Image Compress/1
  Channel/1 -> Video Display/1

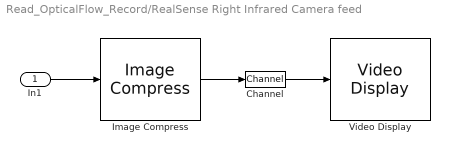
== system Read_OpticalFlow_Record/RealSense Right Infrared Camera feed ==
  In1 : Inport
  Channel : quarc_library/Signal Routing/Channel  channel=5  buffer_size=1
  Image Compress : quarc_library/Image Processing/Generic/Image Compress  algorithm=JPEG  source=Internal dialog parameter  quality=quality  output_dim=-1
  Video Display : quarc_library/Multimedia/Video Display  Tag=Read_OpticalFlow_Record/RealSense Right Infrared Camera feed/Video Display  sample_time=sample_time  use_hardware=on
  wires:
  Image Compress/1 -> Channel/1
  In1/1 -> Image Compress/1
  Channel/1 -> Video Display/1

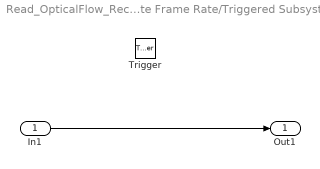
== system Read_OpticalFlow_Record/ Calculate Frame Rate/Triggered Subsystem ==
  In1 : Inport
  Trigger : TriggerPort  VariantControl=Variant
  Out1 : Outport
  wires:
  In1/1 -> Out1/1

== system Read_OpticalFlow_Record/Calculate Frame Rate  /Triggered Subsystem ==
  In1 : Inport
  Trigger : TriggerPort  VariantControl=Variant
  Out1 : Outport
  wires:
  In1/1 -> Out1/1

== system Read_OpticalFlow_Record/Calculate Frame Rate /Triggered Subsystem ==
  In1 : Inport
  Trigger : TriggerPort  VariantControl=Variant
  Out1 : Outport
  wires:
  In1/1 -> Out1/1

== system Read_OpticalFlow_Record/Calculate Frame Rate/Triggered Subsystem ==
  In1 : Inport
  Trigger : TriggerPort  VariantControl=Variant
  Out1 : Outport
  wires:
  In1/1 -> Out1/1

== system Read_OpticalFlow_Record/Calculate Frame Rate /Triggered Subsystem ==
  In1 : Inport
  Trigger : TriggerPort  VariantControl=Variant
  Out1 : Outport
  wires:
  In1/1 -> Out1/1
